simulink model "sf_dcmotor"  (R2025b)
settings: Solver=ode45  StartTime=0.0  StopTime=10  RelTol=1e-3  EnableMultiTasking=on
settings Model: Creator=The MathWorks, Inc.  LastModifiedBy=The MathWorks, Inc.
settings SolverCC: AlgebraicLoopSolver=TrustRegion
settings DataIOCC: LimitDataPoints=on  SaveFormat=Array  ReturnWorkspaceOutputs=off
settings OptimizationCC: ReuseModelBlockBuffer=off  ExpressionDepthLimit=2147483647.0  InitFltsAndDblsToZero=on  LifeSpan=inf
settings DebuggingCC: UnderspecifiedInitializationDetection=Classic  MergeDetectMultiDrivingBlocksExec=none  FcnCallInpInsideContextMsg=warning  UnconnectedInputMsg=warning  UnconnectedOutputMsg=warning  UnconnectedLineMsg=warning  StateNameClashWarn=warning  SFUnexpectedBacktrackingDiag=warning  SFNoUnconditionalDefaultTransitionDiag=warning  SFExecutionAtInitializationDiag=none  ArithmeticOperatorsInVariantConditions=warning
settings HardwareCC: ProdBitPerPointer=32.0  ProdBitPerSizeT=32.0  ProdBitPerPtrDiffT=32.0  ProdLargestAtomicFloat=None  ProdIntDivRoundTo=Undefined  ProdEndianess=Unspecified  ProdWordSize=32.0  ProdHWDeviceType=32-bit Generic
settings ModelReferenceCC: EnableRefExpFcnMdlSchedulingChecks=on  PropagateSignalLabelsOutOfModel=off
settings SFSimCC: SimUseLocalCustomCode=off  SimParseCustomCode=off  CustomCodeUndefinedFunction=UseInterfaceOnly
settings RTWCC: RTWUseLocalCustomCode=off  GPUComputeCapability=3.5  DLArmComputeVersion=19.05
settings CodeAppCC: StateflowObjectComments=on
settings GRTTargetCC: TargetLangStandard=C89/C90 (ANSI)  CombineOutputUpdateFcns=off  GRTInterface=on
settings ConfigComp: CovMetricSettings=dw  CovSaveCumulativeToWorkspaceVar=on  CovSaveSingleToWorkspaceVar=on  CovExternalEMLEnable=off  CovSFcnEnable=off

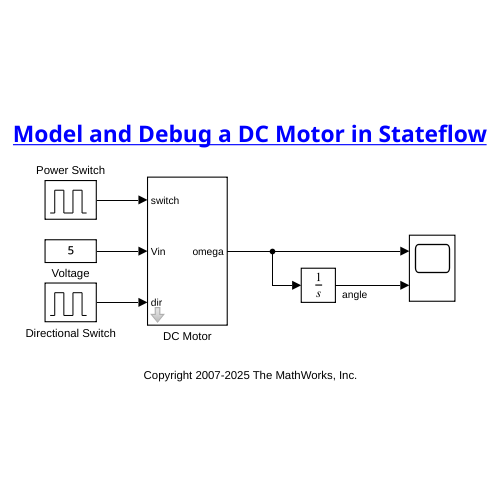
[thumbnail: Simulink's stored preview of the top-level diagram]
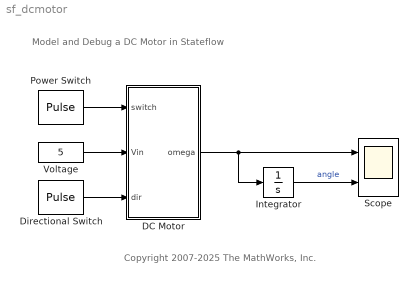
== system sf_dcmotor ==
  note: Copyright 2007-2025 The MathWorks, Inc.
  note: Model and Debug a DC Motor in Stateflow
  DC Motor : Subsystem  mask{R=2.0, L=0.5, Km=.015, Kb=.015, Kf=0.2, J=0.02}
      mask prompts: R "Resistance (Ohms)"; L "Inductance (Henrys)"; Km "Torque Constant"; Kb "EMF Constant"; Kf "Damping Constant"; J "Inertia"
  Directional Switch : DiscretePulseGenerator  PulseType=Time based  Period=1  PulseWidth=50
  Integrator : Integrator
  Power Switch : DiscretePulseGenerator  PulseType=Time based  Period=5  PulseWidth=50  PhaseDelay=2.5
  Scope : Scope  NumInputPorts=2
      settings: ActiveDisplayYMinimum=-0.17861  ActiveDisplayYMaximum=0.14718
  Voltage : Constant  Value=5
  wires:
  Voltage/1 -> DC Motor/2(Vin)
  DC Motor/1(omega) -> Integrator/1, Scope/1
  Integrator/1 -> Scope/2  "angle"
  Directional Switch/1 -> DC Motor/3(dir)
  Power Switch/1 -> DC Motor/1(switch)

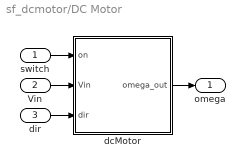
== system sf_dcmotor/DC Motor ==
  switch : Inport
  Vin : Inport  Port=2
  dir : Inport  Port=3
  dcMotor : Stateflow chart  TreatAsAtomicUnit=on
  omega : Outport  VectorParamsAs1DForOutWhenUnconnected=off
  wires:
  switch/1 -> dcMotor/1(on)
  dcMotor/1(omega_out) -> omega/1
  Vin/1 -> dcMotor/2(Vin)
  dir/1 -> dcMotor/3(dir)

== stateflow chart sf_dcmotor/DC Motor/dcMotor ==
  settings: updateMethod=CONTINUOUS  initializeOutput=1
  state powerOn
    state down
      du:
      % Derivatives
      curr_dot = idotCalc(-Vin,curr,omega);
      omega_dot = wdotCalc(curr,omega);
      % Output
      omega_out=omega;
    state up
      du:
      % Derivatives
      curr_dot = idotCalc(Vin,curr,omega);
      omega_dot = wdotCalc(curr,omega);
      % Output
      omega_out=omega;
    (default) -> down [order 2]
    (default) -> up [order 1] : [dir == 1]
    down -> up : [dir==1]
    up -> down : [dir==0]
  state powerOff
    du:
    % Derivatives
    curr_dot = idotCalc(0,curr,omega);
    omega_dot = wdotCalc(curr,omega);
    % Output
    omega_out=omega;
  state der = wdotCalc(i,w) [function]
    (default) -> (junction 17) : {der=Km/J.*i - Kf/J.*w;}
  state der = idotCalc(volts,i,w) [function]
    (default) -> (junction 16) : {der=-R/L.*i - Kb/L.*w + 1.0/L.*volts;}
  (default) -> powerOff : {curr=0;
      | omega=0;}
  powerOn -> powerOff : [~on]
  powerOff -> powerOn : [on]
  data: der function_output double; i function_input double; w function_input double; volts function_input double; der function_output double; i function_input double; w function_input double; curr local double; on input; omega local double; omega_out output double; Vin input double; J parameter double; Kb parameter double; Kf parameter double; Km parameter double; L parameter double; R parameter double; dir input
  data curr settings: updateMethod=SF_CONTINUOUS_TIME_DATA
  data omega settings: updateMethod=SF_CONTINUOUS_TIME_DATA
